simulink model "all_sc_0001_0193"  (R2026a)
settings: Solver=VariableStepAuto  StopTime=40  FixedStep=0.1  MaxStep=.1
model workspace (MAT data in the model file):
  T = [0 0.05 0.1 0.15 0.2 0.25 0.3 0.35 0.4 0.45 0.5 0.55 ... (701 elements, 701x1)]
  U = [3.99594136536 3.99594136536 3.99594136536 3.99594136536 3.99594136536 3.99594136536 3.99594136536 3.99594136536 3.99594136536 3.99594136536 3.99594136536 3.99594136536 ... (701 elements, 701x1)]
undefined symbols (not defined in the file): A, B, C, Dd
(part 3 of 3)

== system all_sc_0001_0193/Subsystem/Layer Recurrent Neural Network 3 layers /Layer 2/Delays 1/FIMWB_133 ==
  Original : Inport
  Result : Outport
  wires:
  Original/1 -> Result/1

== system all_sc_0001_0193/Subsystem/Layer Recurrent Neural Network 3 layers /Layer 2/LW{2,1}/FIMWB_135 ==
  Original : Inport
  Result : Outport
  wires:
  Original/1 -> Result/1

== system all_sc_0001_0193/Subsystem/Layer Recurrent Neural Network 3 layers /Layer 2/LW{2,1}/FIMWB_136 ==
  Original : Inport
  Result : Outport
  wires:
  Original/1 -> Result/1

== system all_sc_0001_0193/Subsystem/Layer Recurrent Neural Network 3 layers /Layer 2/LW{2,1}/FIMWB_137 ==
  Original : Inport
  Result : Outport
  wires:
  Original/1 -> Result/1

== system all_sc_0001_0193/Subsystem/Layer Recurrent Neural Network 3 layers /Layer 2/LW{2,1}/FIMWB_141 ==
  Original : Inport
  Result : Outport
  wires:
  Original/1 -> Result/1

== system all_sc_0001_0193/Subsystem/Layer Recurrent Neural Network 3 layers /Layer 2/LW{2,1}/dotprod1 ==
  In1 : Inport
  In2 : Inport  Port=2
  Dot Product : DotProduct  OutDataTypeStr=Inherit: Inherit via internal rule
  FIMWB_138 : Subsystem  Tag=fimwb.fault.138
  FIMWB_139 : Subsystem  Tag=fimwb.fault.139
  FIMWB_140 : Subsystem  Tag=fimwb.fault.140
  Out1 : Outport  VectorParamsAs1DForOutWhenUnconnected=off
  wires:
  In1/1 -> FIMWB_138/1(Original)
  FIMWB_138/1(Result) -> Dot Product/1
  In2/1 -> FIMWB_139/1(Original)
  FIMWB_139/1(Result) -> Dot Product/2
  Dot Product/1 -> FIMWB_140/1(Original)
  FIMWB_140/1(Result) -> Out1/1

== system all_sc_0001_0193/Subsystem/Layer Recurrent Neural Network 3 layers /Layer 2/purelin/FIMWB_144 ==
  Original : Inport
  Result : Outport
  wires:
  Original/1 -> Result/1

== system all_sc_0001_0193/Subsystem/Layer Recurrent Neural Network 3 layers /Process Input 1/mapminmax/FIMWB_148 ==
  Original : Inport
  Result : Outport
  wires:
  Original/1 -> Result/1

== system all_sc_0001_0193/Subsystem/Layer Recurrent Neural Network 3 layers /Process Input 1/mapminmax/FIMWB_149 ==
  Original : Inport
  Result : Outport
  wires:
  Original/1 -> Result/1

== system all_sc_0001_0193/Subsystem/Layer Recurrent Neural Network 3 layers /Process Input 1/mapminmax/FIMWB_150 ==
  Original : Inport
  Result : Outport
  wires:
  Original/1 -> Result/1

== system all_sc_0001_0193/Subsystem/Layer Recurrent Neural Network 3 layers /Process Input 1/mapminmax/FIMWB_151 ==
  Original : Inport
  Result : Outport
  wires:
  Original/1 -> Result/1

== system all_sc_0001_0193/Subsystem/Layer Recurrent Neural Network 3 layers /Process Output 1/mapminmax_reverse/FIMWB_155 ==
  Original : Inport
  Result : Outport
  wires:
  Original/1 -> Result/1

== system all_sc_0001_0193/Subsystem/Layer Recurrent Neural Network 3 layers /Process Output 1/mapminmax_reverse/FIMWB_156 ==
  Original : Inport
  Result : Outport
  wires:
  Original/1 -> Result/1

== system all_sc_0001_0193/Subsystem/Layer Recurrent Neural Network 3 layers /Process Output 1/mapminmax_reverse/FIMWB_157 ==
  Original : Inport
  Result : Outport
  wires:
  Original/1 -> Result/1

== system all_sc_0001_0193/Subsystem/Layer Recurrent Neural Network 3 layers /Process Output 1/mapminmax_reverse/FIMWB_158 ==
  Original : Inport
  Result : Outport
  wires:
  Original/1 -> Result/1

== system all_sc_0001_0193/Subsystem/Layer Recurrent Neural Network 3 layers /Layer 1/IW{1,1}/dotprod1/FIMWB_085 ==
  Original : Inport
  Result : Outport
  wires:
  Original/1 -> Result/1

== system all_sc_0001_0193/Subsystem/Layer Recurrent Neural Network 3 layers /Layer 1/IW{1,1}/dotprod1/FIMWB_086 ==
  Original : Inport
  Result : Outport
  wires:
  Original/1 -> Result/1

== system all_sc_0001_0193/Subsystem/Layer Recurrent Neural Network 3 layers /Layer 1/IW{1,1}/dotprod1/FIMWB_087 ==
  Original : Inport
  Result : Outport
  wires:
  Original/1 -> Result/1

== system all_sc_0001_0193/Subsystem/Layer Recurrent Neural Network 3 layers /Layer 1/IW{1,1}/dotprod2/FIMWB_089 ==
  Original : Inport
  Result : Outport
  wires:
  Original/1 -> Result/1

== system all_sc_0001_0193/Subsystem/Layer Recurrent Neural Network 3 layers /Layer 1/IW{1,1}/dotprod2/FIMWB_090 ==
  Original : Inport
  Result : Outport
  wires:
  Original/1 -> Result/1

== system all_sc_0001_0193/Subsystem/Layer Recurrent Neural Network 3 layers /Layer 1/IW{1,1}/dotprod2/FIMWB_091 ==
  Original : Inport
  Result : Outport
  wires:
  Original/1 -> Result/1

== system all_sc_0001_0193/Subsystem/Layer Recurrent Neural Network 3 layers /Layer 1/IW{1,1}/dotprod3/FIMWB_093 ==
  Original : Inport
  Result : Outport
  wires:
  Original/1 -> Result/1

== system all_sc_0001_0193/Subsystem/Layer Recurrent Neural Network 3 layers /Layer 1/IW{1,1}/dotprod3/FIMWB_094 ==
  Original : Inport
  Result : Outport
  wires:
  Original/1 -> Result/1

== system all_sc_0001_0193/Subsystem/Layer Recurrent Neural Network 3 layers /Layer 1/IW{1,1}/dotprod3/FIMWB_095 ==
  Original : Inport
  Result : Outport
  wires:
  Original/1 -> Result/1

== system all_sc_0001_0193/Subsystem/Layer Recurrent Neural Network 3 layers /Layer 1/LW{1,1}/dotprod1/FIMWB_105 ==
  Original : Inport
  Result : Outport
  wires:
  Original/1 -> Result/1

== system all_sc_0001_0193/Subsystem/Layer Recurrent Neural Network 3 layers /Layer 1/LW{1,1}/dotprod1/FIMWB_106 ==
  Original : Inport
  Result : Outport
  wires:
  Original/1 -> Result/1

== system all_sc_0001_0193/Subsystem/Layer Recurrent Neural Network 3 layers /Layer 1/LW{1,1}/dotprod1/FIMWB_107 ==
  Original : Inport
  Result : Outport
  wires:
  Original/1 -> Result/1

== system all_sc_0001_0193/Subsystem/Layer Recurrent Neural Network 3 layers /Layer 1/LW{1,1}/dotprod2/FIMWB_109 ==
  Original : Inport
  Result : Outport
  wires:
  Original/1 -> Result/1

== system all_sc_0001_0193/Subsystem/Layer Recurrent Neural Network 3 layers /Layer 1/LW{1,1}/dotprod2/FIMWB_110 ==
  Original : Inport
  Result : Outport
  wires:
  Original/1 -> Result/1

== system all_sc_0001_0193/Subsystem/Layer Recurrent Neural Network 3 layers /Layer 1/LW{1,1}/dotprod2/FIMWB_111 ==
  Original : Inport
  Result : Outport
  wires:
  Original/1 -> Result/1

== system all_sc_0001_0193/Subsystem/Layer Recurrent Neural Network 3 layers /Layer 1/LW{1,1}/dotprod3/FIMWB_113 ==
  Original : Inport
  Result : Outport
  wires:
  Original/1 -> Result/1

== system all_sc_0001_0193/Subsystem/Layer Recurrent Neural Network 3 layers /Layer 1/LW{1,1}/dotprod3/FIMWB_114 ==
  Original : Inport
  Result : Outport
  wires:
  Original/1 -> Result/1

== system all_sc_0001_0193/Subsystem/Layer Recurrent Neural Network 3 layers /Layer 1/LW{1,1}/dotprod3/FIMWB_115 ==
  Original : Inport
  Result : Outport
  wires:
  Original/1 -> Result/1

== system all_sc_0001_0193/Subsystem/Layer Recurrent Neural Network 3 layers /Layer 2/LW{2,1}/dotprod1/FIMWB_138 ==
  Original : Inport
  Result : Outport
  wires:
  Original/1 -> Result/1

== system all_sc_0001_0193/Subsystem/Layer Recurrent Neural Network 3 layers /Layer 2/LW{2,1}/dotprod1/FIMWB_139 ==
  Original : Inport
  Result : Outport
  wires:
  Original/1 -> Result/1

== system all_sc_0001_0193/Subsystem/Layer Recurrent Neural Network 3 layers /Layer 2/LW{2,1}/dotprod1/FIMWB_140 ==
  Original : Inport
  Result : Outport
  wires:
  Original/1 -> Result/1
